simulink model "TF"  (R2023b)
settings: Solver=VariableStepAuto  StartTime=0.0  StopTime=10  RelTol=1e-3
libraries: fl_lib x10, nesl_utility x6, ee_lib x1
settings Model: Creator=g202204960  LastModifiedBy=g202204960
settings OptimizationCC: ReuseModelBlockBuffer=off

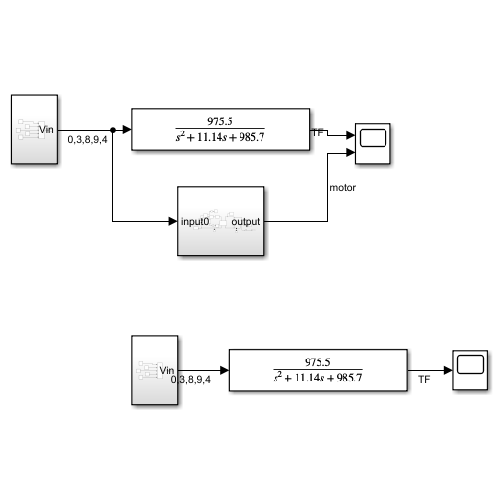
[thumbnail: Simulink's stored preview of the top-level diagram]
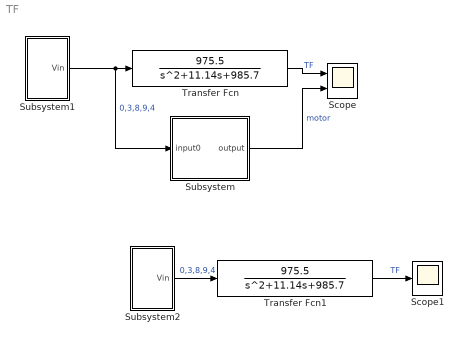
== system TF ==
  Scope : Scope  NumInputPorts=2
  Scope1 : Scope
  Subsystem : Subsystem
  Subsystem1 : Subsystem
  Subsystem2 : Subsystem
  Transfer Fcn : TransferFcn  Numerator=[975.5]  Denominator=[1, 11.14, 985.7]
  Transfer Fcn1 : TransferFcn  Numerator=[975.5]  Denominator=[1, 11.14, 985.7]
  wires:
  Transfer Fcn/1 -> Scope/1  "TF"
  Subsystem/1(output) -> Scope/2  "motor"
  Transfer Fcn1/1 -> Scope1/1  "TF"
  Subsystem1/1(Vin) -> Subsystem/1(input0), Transfer Fcn/1  "0,3,8,9,4"
  Subsystem2/1(Vin) -> Transfer Fcn1/1  "0,3,8,9,4"

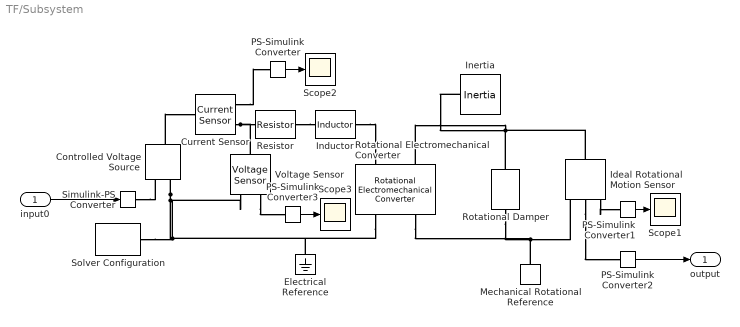
== system TF/Subsystem ==
  input0 : Inport
  Controlled Voltage Source : fl_lib/Electrical/Electrical Sources/Controlled Voltage Source
  Current Sensor : fl_lib/Electrical/Electrical Sensors/Current Sensor
  Electrical Reference : fl_lib/Electrical/Electrical Elements/Electrical Reference
  Ideal Rotational Motion Sensor : fl_lib/Mechanical/Mechanical Sensors/Ideal Rotational Motion Sensor  reference=foundation.enum.MeasurementReference.difference  acceleration_port=false  velocity_port=true  position_port=true  wrap_angle=false  offset=0 rad
  Inductor : ee_lib/Passive/Inductor  l=0.1 H  enable_L_tol=0  L_tol=20  tol_distribution=1  nSigma=4  r=0 Ohm  g=1e-9 1/Ohm  enable_operating_limits=0  operating_limit_action=2  max_working_current=1 A  power_rating=1 W  enable_faults=ee.enum.enable.no  fault_action=simscape.enum.assert.action.none  lambdaPercent=50  k_faulted=0.9999  turnsShort=0  openCct=0  groundShort=0  groundShortG=0 1/Ohm  tau_fault=1e-3 s  fault_trigger=ee.enum.faults.faultTrigger.temporal  t_fault=1 s  max_permissible_voltage=100 V  n_fail_on_voltage=1  max_permissible_current=1 A  t_fail_on_current=1 s  i_L_specify=off  i_L_priority=High  i_L=0 A  i_L_nominal_specify=off  i_L_nominal_unit=A  i_L_nominal_value=1
  Inertia : fl_lib/Mechanical/Rotational Elements/Inertia  inertia=0.01 kg*m^2  num_ports=foundation.enum.numPorts2.one  w_specify=off  w_priority=High  w=0 rad/s  w_nominal_specify=off  w_nominal_unit=rad/s  w_nominal_value=1  t_specify=off  t_priority=None  t=0 N*m  t_nominal_specify=off  t_nominal_unit=N*m  t_nominal_value=1
  Mechanical Rotational Reference : fl_lib/Mechanical/Rotational Elements/Mechanical Rotational Reference
  PS-Simulink Converter{,1..3} (4 alike) : nesl_utility/PS-Simulink Converter  PhysicalDomain=network_engine_domain  SubClassName=ps_output  LeftPortType=input  RightPortType=output  PseudoPeriodic=off  Frequencies=[]  VectorFormat=inherit  Unit=inherit  AffineConversion=off
  Resistor : fl_lib/Electrical/Electrical Elements/Resistor  R=1 Ohm  i_specify=off  i_priority=None  i=0 A  i_nominal_specify=off  i_nominal_unit=A  i_nominal_value=1  v_specify=off  v_priority=None  v=0 V  v_nominal_specify=off  v_nominal_unit=V  v_nominal_value=1
  Rotational Electromechanical Converter : fl_lib/Electrical/Electrical Elements/Rotational Electromechanical Converter  K=1 V*s/rad  i_specify=off  i_priority=None  i=0 A  i_nominal_specify=off  i_nominal_unit=A  i_nominal_value=1  v_specify=off  v_priority=None  v=0 V  v_nominal_specify=off  v_nominal_unit=V  v_nominal_value=1  t_specify=off  t_priority=None  t=0 N*m  t_nominal_specify=off  t_nominal_unit=N*m  t_nominal_value=1  w_specify=off  w_priority=None  w=0 rad/s  w_nominal_specify=off  w_nominal_unit=rad/s  w_nominal_value=1
  Rotational Damper : fl_lib/Mechanical/Rotational Elements/Rotational Damper  D=0.01 N*m*s/rad  w_specify=off  w_priority=None  w=0 rad/s  w_nominal_specify=off  w_nominal_unit=rad/s  w_nominal_value=1  t_specify=off  t_priority=None  t=0 N*m  t_nominal_specify=off  t_nominal_unit=N*m  t_nominal_value=1
  Scope1 : Scope
  Scope2 : Scope
  Scope3 : Scope
  Simulink-PS Converter : nesl_utility/Simulink-PS Converter  PhysicalDomain=network_engine_domain  SubClassName=ps_input  LeftPortType=input  RightPortType=output  PseudoPeriodic=off  Frequencies=[]  NoiseDistribution=none  NoiseParameters=[]  Unit=1  AffineConversion=off  FilteringAndDerivatives=provide  SimscapeFilterOrder=1  InputFilterTimeConstant=0.001  UdotUserProvided=0
  Solver Configuration : nesl_utility/Solver Configuration  PhysicalDomain=network_engine_domain  SubClassName=solver  LeftPortType=input  RightPortType=generic  Tones=[]  Harmonics=[]  SimulateNoise=off  Profile=off  UseLocalSampling=off  EnableSwitchedLinearOptims=on  FrequencyDomain=off  UseCCode=off  RelTol=0.001  AbsTol=0.001  MinStep=1e-09  ToWorkspace=off  RevertToSquareIcSolve=off  NumHomotopyIterations=100  PhasorMode=off  PhasorModeNumHarmonics=1  ConsistencySolver=NEWTON_XTOL_AFTER_FTOL  IndexReductionMethod=DerivativeReplacement  DoDC=off  ResidualTolerance=1e-09  ConsistencyTolSource=GLOBAL  ConsistencyAbsTol=0.001  ConsistencyRelTol=0.001  ConsistencyTolFactor=0.001  UseLocalSolver=off  LocalSolverChoice=NE_BACKWARD_EULER_ADVANCER  ResolveIndetEquations=on  FunctionEvalNumThread=1  LocalSolverSampleTime=0.001  DoFixedCost=off  MaxNonlinIter=3  MaxModeIter=2  ComputeImpulses=off  ImpulseIterations=2  LinearAlgebra=auto  LinearAlgebraNumThread=0  EquationFormulation=NE_TIME_EF  DelaysMemoryBudget=1024  AutomaticFiltering=on  FilteringTimeConstant=0.001  PartitionStorageMethod=AS_NEEDED  PartitionMemoryBudget=1024  PartitionMethod=ROBUST  MultibodyUseLocalSolver=off  MultibodyLocalSolverChoice=ODE1  MultibodyLocalSolverSampleTime=0.001
  Voltage Sensor : fl_lib/Electrical/Electrical Sensors/Voltage Sensor
  output : Outport
  wires:
  PS-Simulink Converter1/1 -> Scope1/1
  PS-Simulink Converter/1 -> Scope2/1
  PS-Simulink Converter3/1 -> Scope3/1
  input0/1 -> Simulink-PS Converter/1
  PS-Simulink Converter2/1 -> output/1
  connections:
  Resistor/LConn1 -- Current Sensor/RConn2 -- Voltage Sensor/LConn1
  Controlled Voltage Source/RConn2 -- Voltage Sensor/RConn2 -- Solver Configuration/RConn1 -- Rotational Electromechanical Converter/RConn1 -- Electrical Reference/LConn1
  Simulink-PS Converter/RConn1 -- Controlled Voltage Source/RConn1
  Mechanical Rotational Reference/LConn1 -- Rotational Electromechanical Converter/RConn2 -- Rotational Damper/RConn1 -- Ideal Rotational Motion Sensor/RConn1
  Rotational Damper/LConn1 -- Rotational Electromechanical Converter/LConn2 -- Inertia/LConn1 -- Ideal Rotational Motion Sensor/LConn1
  Ideal Rotational Motion Sensor/RConn2 -- PS-Simulink Converter2/LConn1
  Controlled Voltage Source/LConn1 -- Current Sensor/LConn1
  Inductor/RConn1 -- Rotational Electromechanical Converter/LConn1
  Current Sensor/RConn1 -- PS-Simulink Converter/LConn1
  Resistor/RConn1 -- Inductor/LConn1
  Voltage Sensor/RConn1 -- PS-Simulink Converter3/LConn1
  Ideal Rotational Motion Sensor/RConn3 -- PS-Simulink Converter1/LConn1

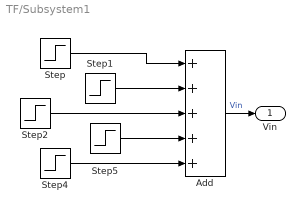
== system TF/Subsystem1 ==
  Add : Sum  Inputs=+++++
  Step : Step  Time=0  After=3  SampleTime=0.01  ZeroCross=off
  Step1 : Step  Time=3  After=5  SampleTime=0.01  ZeroCross=off
  Step2 : Step  Time=5  After=7  SampleTime=0.01  ZeroCross=off
  Step4 : Step  Time=5  After=-6  SampleTime=0.01  ZeroCross=off
  Step5 : Step  Time=7  After=-5  SampleTime=0.01  ZeroCross=off
  Vin : Outport
  wires:
  Step/1 -> Add/1
  Add/1 -> Vin/1  "Vin"
  Step2/1 -> Add/3
  Step5/1 -> Add/4
  Step1/1 -> Add/2
  Step4/1 -> Add/5

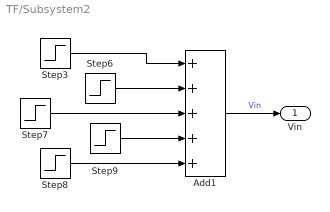
== system TF/Subsystem2 ==
  Add1 : Sum  Inputs=+++++
  Step3 : Step  Time=0  After=3  SampleTime=0.01  ZeroCross=off
  Step6 : Step  Time=3  After=5  SampleTime=0.01  ZeroCross=off
  Step7 : Step  Time=5  After=7  SampleTime=0.01  ZeroCross=off
  Step8 : Step  Time=5  After=-6  SampleTime=0.01  ZeroCross=off
  Step9 : Step  Time=7  After=-5  SampleTime=0.01  ZeroCross=off
  Vin : Outport
  wires:
  Add1/1 -> Vin/1  "Vin"
  Step6/1 -> Add1/2
  Step3/1 -> Add1/1
  Step7/1 -> Add1/3
  Step8/1 -> Add1/5
  Step9/1 -> Add1/4
